simulink model "mimo_test2"  (R2025b)
settings: Solver=ode8  StartTime=0.0  StopTime=10.0  FixedStep=0.01  RelTol=1e-3
settings Model: Creator=MehrSystem  LastModifiedBy=MehrSystem

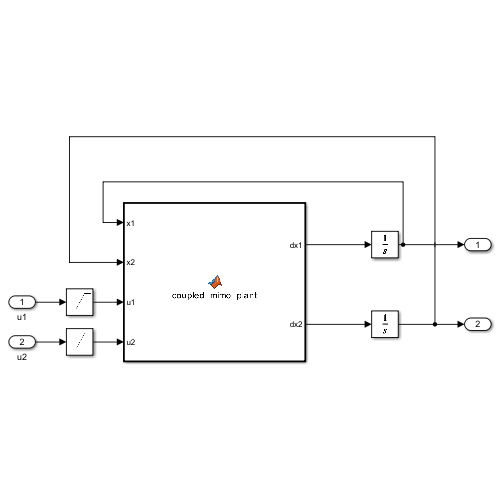
[thumbnail: Simulink's stored preview of the top-level diagram]
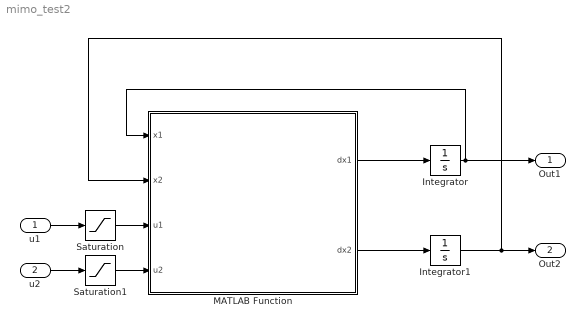
== system mimo_test2 ==
  u1 : Inport
  u2 : Inport  Port=2
  Integrator : Integrator
  Integrator1 : Integrator
  MATLAB Function : MATLAB Function  TreatAsAtomicUnit=on
  Saturation : Saturate  UpperLimit=0.7  LowerLimit=-0.9
  Saturation1 : Saturate  UpperLimit=0.95  LowerLimit=-0.85
  Out1 : Outport
  Out2 : Outport  Port=2
  wires:
  MATLAB Function/1(dx1) -> Integrator/1
  MATLAB Function/2(dx2) -> Integrator1/1
  Integrator/1 -> MATLAB Function/1(x1), Out1/1
  Integrator1/1 -> MATLAB Function/2(x2), Out2/1
  u1/1 -> Saturation/1
  u2/1 -> Saturation1/1
  Saturation/1 -> MATLAB Function/3(u1)
  Saturation1/1 -> MATLAB Function/4(u2)

== matlab function mimo_test2/MATLAB Function ==
  data: x1 input; dx1 output; x2 input; u1 input; u2 input; dx2 output
function [dx1, dx2] = coupled_mimo_plant(x1, x2, u1, u2)
    % System parameters for a stable coupled dynamic system
    a11 = -0.5;
    a12 = 0.2;
    a21 = 0.1;
    a22 = -0.3;
    
    b1 = 1.0;
    b2 = 1.5;

    % Differential equations
    dx1 = a11 * x1 + a12 * x2 + b1 * u1;
    dx2 = a21 * x1 + a22 * x2 + b2 * u2;
end
